simulink model "Comparaciones"  (R2026b)
settings: Solver=VariableStepAuto  StopTime=3
values from neighbouring files (symbols this model uses):
  g = 9.80665    [coeficientes.m]
  T_amb = 20    [coeficientes.m]
settings Model: Creator=admin  LastModifiedBy=lamun
settings SimscapeCC: SimscapeNominalValues="[{\"value\":\"1\",\"unit\":\"A\"},{\"value\":\"1\",\"unit\":\"bar\"},{\"value\":\"1\",\"unit\":\"cm^2\"},{\"value\":\"1\",\"unit\":\"cm^3/s\"},{\"value\":\"1\",\"unit\":\"kJ/kg\"},{\"value\":\"1\",\"unit\":\"kW\"},{\"value\":\"1\",\"unit\":\"l\"},{\"value\":\"1\",\"unit\":\"N\"},{\"value\":\"1\",\"unit\":\"N*m\"},{\"value\":\"1\",\"unit\":\"V\"},{\"value\":\"0.001\",\"unit\":\"Wb\"}]"  SimscapeUseEnergyAccounting=off

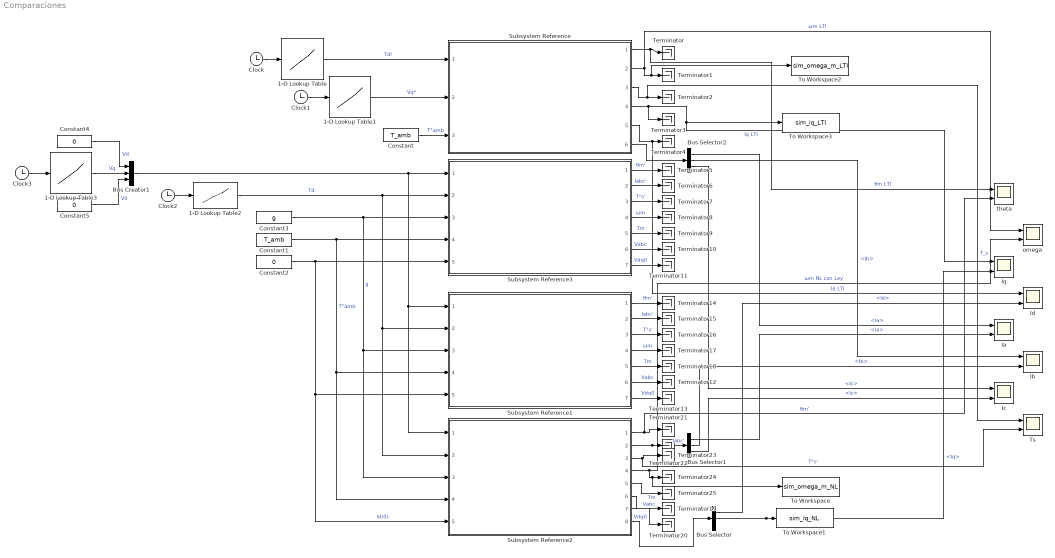
== system Comparaciones ==
  1-D Lookup Table : Lookup_n-D  NumberOfTableDimensions=1  BreakpointsForDimension1=[0.0, 0.1, 0.101, 0.3, 0.301, 0.5, 0.501, 0.7, 0.701, 0.9, 0.901, 1.1, 1.101, 1.3, 1.301, 1.5, 1.501, 1.7, 1.701, 1.9, 1.901, 2.0]  Table=[0.0, 0.0, 0.0, 0.0, 6.28, 6.28, -6.28, -6.28, -6.28, -6.28, 0.0, 0.0, 0.0, 0.0, 6.28, 6.28, -6.28, -6.28, 0.0, 0.0, 0.0, 0.0]  InternalRulePriority=Speed  RndMeth=Simplest
  1-D Lookup Table1 : Lookup_n-D  NumberOfTableDimensions=1  BreakpointsForDimension1=[0.0, 0.1, 0.101, 0.3, 0.301, 0.5, 0.501, 0.7, 0.701, 0.9, 0.901, 1.1, 1.101, 1.3, 1.301, 1.5, 1.501, 1.7, 1.701, 1.9, 1.901, 2.0]  Table=[0.0, 0.0, 19.596, 19.596, 19.596, 19.596, 19.596, 19.596, 0.0, 0.0, 0.0, 0.0, -19.596, -19.596, -19.596, -19.596, -19.596, -19.596, 0.0, 0.0, 0.0, 0.0]  InternalRulePriority=Speed  RndMeth=Simplest
  1-D Lookup Table2 : Lookup_n-D  NumberOfTableDimensions=1  BreakpointsForDimension1=[0.0, 0.1, 0.101, 0.3, 0.301, 0.5, 0.501, 0.7, 0.701, 0.9, 0.901, 1.1, 1.101, 1.3, 1.301, 1.5, 1.501, 1.7, 1.701, 1.9, 1.901, 2.0]  Table=[0.0, 0.0, 0.0, 0.0, 6.28, 6.28, -6.28, -6.28, -6.28, -6.28, 0.0, 0.0, 0.0, 0.0, 6.28, 6.28, -6.28, -6.28, 0.0, 0.0, 0.0, 0.0]  InternalRulePriority=Speed  RndMeth=Simplest
  1-D Lookup Table3 : Lookup_n-D  NumberOfTableDimensions=1  BreakpointsForDimension1=[0.0, 0.1, 0.101, 0.3, 0.301, 0.5, 0.501, 0.7, 0.701, 0.9, 0.901, 1.1, 1.101, 1.3, 1.301, 1.5, 1.501, 1.7, 1.701, 1.9, 1.901, 2.0]  Table=[0.0, 0.0, 19.596, 19.596, 19.596, 19.596, 19.596, 19.596, 0.0, 0.0, 0.0, 0.0, -19.596, -19.596, -19.596, -19.596, -19.596, -19.596, 0.0, 0.0, 0.0, 0.0]  InternalRulePriority=Speed  RndMeth=Simplest
  Bus Creator1 : BusCreator  Inputs=3
  Bus Selector : BusSelector  OutputSignals=Id,Iq,I0
  Bus Selector1 : BusSelector  OutputSignals=Ia,Ib,Ic
  Bus Selector2 : BusSelector  OutputSignals=Ia,Ib,Ic
  Clock{,1..3} (4 alike) : Clock
  Constant : Constant  Value=T_amb
  Constant1 : Constant  Value=T_amb
  Constant2 : Constant  Value=0
  Constant3 : Constant  Value=g
  Constant4 : Constant  Value=0
  Constant5 : Constant  Value=0
  Ia : Scope  NumInputPorts=2
      settings: Title=Comparación Corrientes Ia  ActiveDisplayYMinimum=-15.884839257565949  ActiveDisplayYMaximum=15.842213864627638  YLabel=Corriente Ia  DataLoggingVariableName=ScopeData3
  Ib : Scope  NumInputPorts=2
      settings: Title=Comparación Corrientes Ib  ActiveDisplayYMinimum=-15.786152009863155  ActiveDisplayYMaximum=16.405646746971225  YLabel=Corriente Ib  DataLoggingVariableName=ScopeData4
  Ic : Scope  NumInputPorts=2
      settings: Title=Comparación Corrientes Ic  ActiveDisplayYMinimum=-16.4512604006654  ActiveDisplayYMaximum=15.66373388849809  YLabel=Corriente Ic  DataLoggingVariableName=ScopeData5
  Id : Scope  NumInputPorts=2
      settings: Title=Comparación Corrientes Viruales Id  ActiveDisplayYMinimum=-5  ActiveDisplayYMaximum=5  YLabel=Corriente Virtual Id  DataLoggingVariableName=ScopeData2
  Iq : Scope  NumInputPorts=2
      settings: Title=Comparación Corrientes Viruales Iq  ActiveDisplayYMinimum=-16.431377285300282  ActiveDisplayYMaximum=16.747750319569413  YLabel=Corriente Virtual Iq
  Subsystem Reference : Subsystem  ReferencedSubsystem=Modelo_LTI_Aumentado
  Subsystem Reference1 : Subsystem  ReferencedSubsystem=Modelo_LeyDeControlMinima
  Subsystem Reference2 : Subsystem  ReferencedSubsystem=Modelo_LeyDeControlMinima_Complementaria
  Subsystem Reference3 : Subsystem  ReferencedSubsystem=SistemaNL
  Terminator{,1..25} (26 alike) : Terminator
  To Workspace : ToWorkspace  VariableName=sim_omega_m_NL  SaveFormat=Timeseries  SampleTime=-1
  To Workspace1 : ToWorkspace  VariableName=sim_Iq_NL  SaveFormat=Timeseries  SampleTime=-1
  To Workspace2 : ToWorkspace  VariableName=sim_omega_m_LTI  SaveFormat=Timeseries  SampleTime=-1
  To Workspace3 : ToWorkspace  VariableName=sim_iq_LTI  SaveFormat=Timeseries  SampleTime=-1
  Ts : Scope  NumInputPorts=2
      settings: Title=Comparación de Temperaturas del Estator  ActiveDisplayYMinimum=-2.5307458749722405  ActiveDisplayYMaximum=22.776712874750167  YLabel=Temperatura del estator  DataLoggingVariableName=ScopeData6
  omega : Scope  NumInputPorts=2
      settings: Title=Comparación de Velocidades Angulares  ActiveDisplayYMinimum=-557.25917465100747  ActiveDisplayYMaximum=528.676263540643  YLabel=Velocidad Angular [rad/s]
  theta : Scope  NumInputPorts=2
      settings: Title=Comparación de Posiciones Angulares  ActiveDisplayYMinimum=-57.419430866655254  ActiveDisplayYMaximum=269.428234156848  YLabel=Posición Angular [rad]  DataLoggingVariableName=ScopeData7
  wires:
  Clock/1 -> 1-D Lookup Table/1
  Clock1/1 -> 1-D Lookup Table1/1
  Constant/1 -> Subsystem Reference/3  "T°amb"
  Subsystem Reference/1 -> theta/1, Terminator/1  "θm LTI"
  Subsystem Reference/2 -> To Workspace2/1, Terminator1/1, omega/1  "ωm LTI"
  Subsystem Reference/3 -> Ts/1, Terminator2/1  "T_s"
  Subsystem Reference/4 -> Terminator3/1, Iq/1, To Workspace3/1  "Iq LTI"
  Subsystem Reference/5 -> Id/1, Terminator4/1  "Id LTI"
  Constant1/1 -> Subsystem Reference1/4, Subsystem Reference2/4, Subsystem Reference3/4  "T°amb"
  Constant2/1 -> Subsystem Reference1/5, Subsystem Reference2/5, Subsystem Reference3/5  "Id(0)"
  Subsystem Reference3/1 -> Terminator5/1  "θm'"
  Subsystem Reference3/2 -> Terminator6/1  "Iabc'"
  Subsystem Reference3/3 -> Terminator7/1  "T°s'"
  Subsystem Reference3/4 -> Terminator8/1  "ωm"
  Subsystem Reference3/5 -> Terminator9/1  "Tm"
  Subsystem Reference3/6 -> Terminator10/1  "Vabc"
  Subsystem Reference3/7 -> Terminator11/1  "Vdq0"
  Constant3/1 -> Subsystem Reference2/3, Subsystem Reference1/3, Subsystem Reference3/3  "g"
  1-D Lookup Table3/1 -> Bus Creator1/2  "Vq"
  Clock3/1 -> 1-D Lookup Table3/1
  Clock2/1 -> 1-D Lookup Table2/1
  1-D Lookup Table2/1 -> Subsystem Reference2/2, Subsystem Reference1/2, Subsystem Reference3/2  "Td"
  Constant4/1 -> Bus Creator1/1  "Vd"
  Constant5/1 -> Bus Creator1/3  "V0"
  Bus Creator1/1 -> Subsystem Reference2/1, Subsystem Reference1/1, Subsystem Reference3/1
  1-D Lookup Table1/1 -> Subsystem Reference/2  "Vq*"
  1-D Lookup Table/1 -> Subsystem Reference/1  "Tdl"
  Subsystem Reference1/4 -> Terminator17/1  "ωm"
  Subsystem Reference1/2 -> Terminator15/1  "Iabc'"
  Subsystem Reference1/5 -> Terminator18/1  "Tm"
  Subsystem Reference1/6 -> Terminator12/1  "Vabc"
  Subsystem Reference1/1 -> Terminator14/1  "θm'"
  Subsystem Reference1/7 -> Terminator13/1  "Vdq0"
  Subsystem Reference1/3 -> Terminator16/1  "T°s'"
  Subsystem Reference2/4 -> To Workspace/1, Terminator24/1, omega/2  "ωm NL con Ley"
  Subsystem Reference2/2 -> Terminator22/1, Bus Selector1/1  "Iabc'"
  Subsystem Reference2/5 -> Terminator25/1  "Tm"
  Subsystem Reference2/6 -> Terminator19/1  "Vabc"
  Subsystem Reference2/1 -> theta/2, Terminator21/1  "θm'"
  Subsystem Reference2/7 -> Terminator20/1  "Vdq0"
  Subsystem Reference2/3 -> Ts/2, Terminator23/1  "T°s'"
  Subsystem Reference2/8 -> Bus Selector/1
  Bus Selector/2 -> Iq/2, To Workspace1/1  "<Iq>"
  Bus Selector/1 -> Id/2  "<Id>"
  Bus Selector1/1 -> Ia/2  "<Ia>"
  Subsystem Reference/6 -> Bus Selector2/1
  Bus Selector2/1 -> Ia/1  "<Ia>"
  Bus Selector2/2 -> Ib/1  "<Ib>"
  Bus Selector1/2 -> Ib/2  "<Ib>"
  Bus Selector2/3 -> Ic/1  "<Ic>"
  Bus Selector1/3 -> Ic/2  "<Ic>"
